simulink subsystem "DABPrimaryMOSFETDevice"  (R2026a)
settings: Solver=VariableStepAuto
libraries: ConverterLibrary x1
Description:
  | MOSFET Model device with an energy-conserving thermal coupling: the computed loss is injected as a heat flow into a Simscape junction thermal mass. Built from DABPrimaryMOSFETDevice.
settings Model: Creator=vsolaise  LastModifiedBy=vsolaise

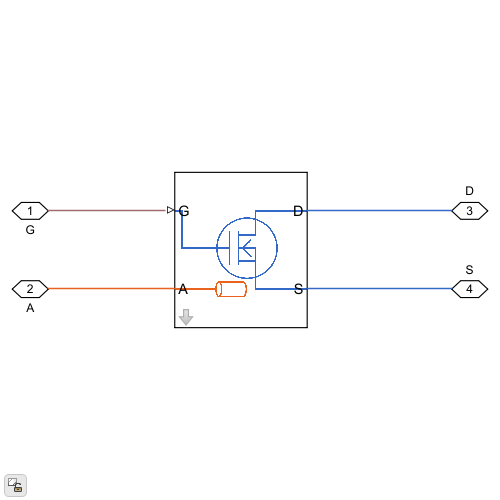
[thumbnail: Simulink's stored preview of the top-level diagram]
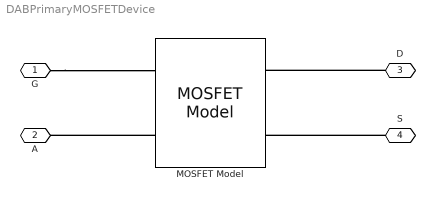
== system DABPrimaryMOSFETDevice ==
  MOSFET Model : ConverterLibrary/Components/MOSFET Model  Vth=DAB.SwitchPri.Vth V  Von_data=DAB.SwitchPri.Von_data V  Tj=DAB.SwitchPri.Tj degC  Iout_data=DAB.SwitchPri.Iout_data A  Iout_data_loss=DAB.SwitchPri.Iout_data_loss A  Tj_loss=DAB.SwitchPri.Tj_loss degC  Eoff_data=DAB.SwitchPri.Eoff_data J  Eon_data=DAB.SwitchPri.Eon_data J  Voff=DAB.SwitchPri.Voff V  Soft_Switching_Flag=on  Tj_diode=DAB.SwitchPri.diode_TjVec degC  If_data=DAB.SwitchPri.diode_IfVec A  Vf_data=DAB.SwitchPri.diode_VfMat V  thermal_resistance=DAB.SwitchPri.R K/W  thermal_mass=DAB.SwitchPri.junction_thermal_mass J/K  Tj0=DAB.simTempPri degC  Goff=DAB.SwitchPri.diode_Goff S  Rds=DAB.SwitchPri.Rds Ohm  GdsOff=DAB.SwitchPri.Goff S
      settings: SourceProductName=Simscape Power Converter Components
  G : PMIOPort  Side=Left
  A : PMIOPort  Port=2  Side=Left
  D : PMIOPort  Port=3  Side=Right
  S : PMIOPort  Port=4  Side=Right
  connections:
  D/RConn1 -- MOSFET Model/RConn1
  S/RConn1 -- MOSFET Model/RConn2
  G/RConn1 -- MOSFET Model/LConn1
  MOSFET Model/LConn2 -- A/RConn1
